simulink model "W06_7_front"  (R2024b)
settings: Solver=ode4  StartTime=0  StopTime=150  FixedStep=h  RelTol=1e-3
InitFcn:
  | addpath(fullfile(fileparts(fileparts(fileparts(get_param(bdroot, 'FileName')))), '_tools'), fileparts(get_param(bdroot, 'FileName'))); run_alone('W06', bdroot);
StopFcn:
  | W06_plot;
values from neighbouring files (symbols this model uses):
  animate = 1    [W06_0_setup.m]    (also in W06_1_point_run.m = 0; W06_2_sway_run.m = 0; W06_3_thrust_run.m = 0; W06_4_stop_run.m = 0)
  berth_E = 1.2    [W06_0_setup.m]
  berth_N = 40    [W06_0_setup.m]
  beta_c = pi/2    (= 1.57079632679)    [W06_0_setup.m]    (also in W06_4_stop_run.m = V.beta_c)
  Binv = inv(B)    [W06_0_setup.m]
  bow = [l_f, k_bow, n_bow_max]    [W06_0_setup.m]
  h = 0.02    [W06_0_setup.m]
  k_bow = cfg.k_bow    [W06_0_setup.m]
  k_neg = cfg.k_neg    [W06_0_setup.m]
  k_pos = cfg.k_pos    [W06_0_setup.m]
  Kb = 1    [W06_0_setup.m]
  Kd = 100    [W06_0_setup.m]
  Ki_u = 200    [W06_0_setup.m]
  Ki_v = 120    [W06_0_setup.m]
  Kp = 300    [W06_0_setup.m]
  Kp_pos = 0.30    (= 0.3)    [W06_0_setup.m]    (also in W06_4_stop_run.m = V.Kp_pos)
  Kp_u = 200    [W06_0_setup.m]
  Kp_v = 150    [W06_0_setup.m]
  mp = 25    [W06_0_setup.m]
  n_bow_max = cfg.n_bow_max    [W06_0_setup.m]    (also in W06_1_point_run.m = V.n_bow_max)
  n_max = cfg.n_max    [W06_0_setup.m]
  N_max = 2*y_pont*min(T_max, -T_min)    [W06_0_setup.m]
  n_min = cfg.n_min    [W06_0_setup.m]
  psi_tol = deg2rad(5)    [W06_0_setup.m]
  R_app = 1.5    [W06_0_setup.m]
  R_berth = 0.40    (= 0.4)    [W06_0_setup.m]
  r_tol = deg2rad(1.0)    [W06_0_setup.m]
  rp = [0.05 0 -0.35]'    [W06_0_setup.m]
  stand_off = 7    [W06_0_setup.m]
  u_lim = 0.80    (= 0.8)    [W06_0_setup.m]
  V_c = 0    [W06_0_setup.m]    (also in W06_4_stop_run.m = V.V_c)
  v_lim = 0.35    [W06_0_setup.m]
  v_tol = 0.05    [W06_0_setup.m]
  x0 = zeros(12,1)    [W06_0_setup.m]
  X_max = 120    [W06_0_setup.m]    (also in W06_plot.m = base_var('X_max', 120))
  Y_max = min(abs(T_min)/(l_f/(2*y_pont)), F_B_max)    [W06_0_setup.m]    (also in W06_plot.m = base_var('Y_max', 35.13))
settings Model: Creator=admin  LastModifiedBy=admin
settings DataIOCC: ReturnWorkspaceOutputs=off

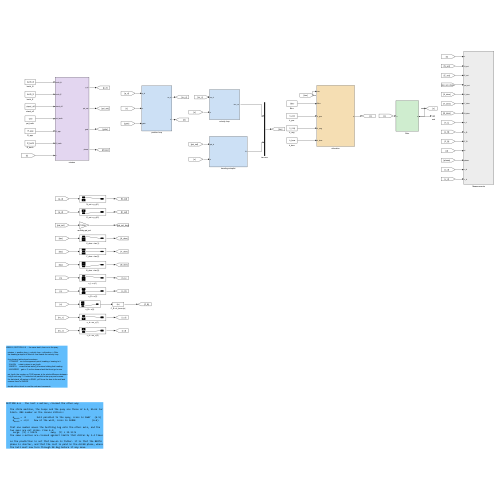
[thumbnail: Simulink's stored preview of the top-level diagram]
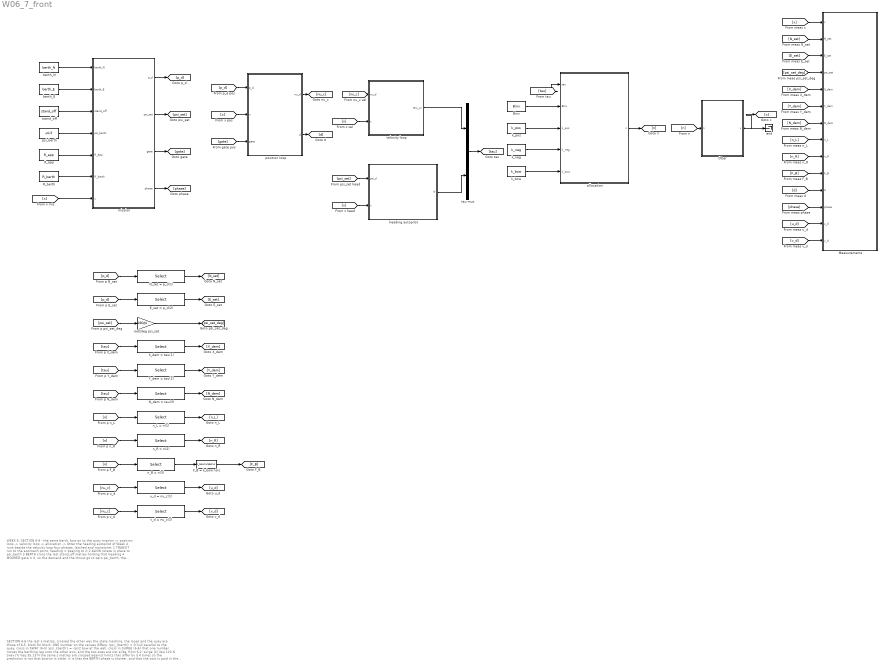
== system W06_7_front ==
  note: WEEK 6, SECTION 6-6  -  the same berth, bow on to the quay
      |
      |    mission -> position loop -> velocity loop -> allocation -> Otter
      |    the heading autopilot of Week 4 runs beside the velocity loop
      |
      |    four phases, latched and monotone:
      |      1 TRANSIT   run to the approach point, heading = bearing to it
      |      2 ALIGN     rotate in place to psi_berth
      |      3 BERTH     cross the last stand_off metres holding that heading
      |      4 MOORED    gate = 0, so the demand and the thrust go to zero
      |
      |    psi_berth, the number on THIS canvas, is the whole difference between
      |    rung 5 and rung 7: 0 holds the hull parallel to the quay and crosses
      |    the last stand_off metres in SWAY, -pi/2 turns the bow to the wall and
      |    crosses them in SURGE
      |
      |    double-click a block to read its code and comments
  note: SECTION 6-6   the last s metres, crossed the other way
      |
      |    the state machine, the loops and the quay are those of 6-5, block for
      |    block. ONE number on the canvas differs:
      |
      |      \psi_{berth} =  0        hull parallel to the quay, cross in SWAY   (6-5)
      |      \psi_{berth} = -\pi/2    bow at the wall, cross in SURGE            (6-6)
      |
      |    that one number moves the berthing leg onto the other axis, and the
      |    two axes are not alike. from 6-2:
      |      surge  |X| \leq 120 N          sway  |Y| \leq 35.13 N
      |    the same s metres are crossed against limits that differ by 3.4 times
      |
      |    so the prediction is not that bow-on is tidier. it is that the BERTH
      |    phase is shorter, and that the cost is paid in the ALIGN phase, where
      |    the hull must now turn through 90 deg before it may move
  Binv : Constant  Value=Binv
  E_set = p_d(2) : Selector  InputPortWidth=2  IndexOptions=Index vector (dialog)  Indices=2  OutputSizes=1
  F_B = k_bow n|n| : Fcn  Expr=k_bow*u*abs(u)
  Measurements : Subsystem
  N_dem = tau(3) : Selector  InputPortWidth=3  IndexOptions=Index vector (dialog)  Indices=3  OutputSizes=1
  N_set = p_d(1) : Selector  InputPortWidth=2  IndexOptions=Index vector (dialog)  Indices=1  OutputSizes=1
  Otter : Subsystem
  R_app : Constant  Value=R_app
  R_berth : Constant  Value=R_berth
  X_dem = tau(1) : Selector  InputPortWidth=3  IndexOptions=Index vector (dialog)  Indices=1  OutputSizes=1
  Y_dem = tau(2) : Selector  InputPortWidth=3  IndexOptions=Index vector (dialog)  Indices=2  OutputSizes=1
  allocation : Subsystem
  berth_E : Constant  Value=berth_E
  berth_N : Constant  Value=berth_N
  end : Terminator
  heading autopilot : Subsystem
  k_bow : Constant  Value=k_bow
  k_neg : Constant  Value=k_neg
  k_pos : Constant  Value=k_pos
  mission : Subsystem
  n_B = n(3) : Selector  InputPortWidth=3  IndexOptions=Index vector (dialog)  Indices=3  OutputSizes=1
  n_L = n(1) : Selector  InputPortWidth=3  IndexOptions=Index vector (dialog)  Indices=1  OutputSizes=1
  n_R = n(2) : Selector  InputPortWidth=3  IndexOptions=Index vector (dialog)  Indices=2  OutputSizes=1
  position loop : Subsystem
  psi_berth : Constant  Value=-pi/2
  rad2deg psi_set : Gain  Gain=180/pi
  stand_off : Constant  Value=stand_off
  tau mux : Mux  Inputs=2
  u_d = nu_c(1) : Selector  InputPortWidth=2  IndexOptions=Index vector (dialog)  Indices=1  OutputSizes=1
  v_d = nu_c(2) : Selector  InputPortWidth=2  IndexOptions=Index vector (dialog)  Indices=2  OutputSizes=1
  velocity loop : Subsystem
  wires:
  berth_N/1 -> mission/1(berth_N)
  berth_E/1 -> mission/2(berth_E)
  stand_off/1 -> mission/3(stand_off)
  psi_berth/1 -> mission/4(psi_berth)
  R_app/1 -> mission/5(R_app)
  R_berth/1 -> mission/6(R_berth)
  [x] -> mission/7(x)
  mission/1(p_d) -> [p_d]
  mission/2(psi_set) -> [psi_set]
  mission/3(gate) -> [gate]
  mission/4(phase) -> [phase]
  [p_d] -> position loop/1(p_d)
  [x] -> position loop/2(x)
  [gate] -> position loop/3(gate)
  position loop/2(d) -> [d]
  position loop/1(nu_d) -> [nu_c]
  [nu_c] -> velocity loop/1(nu_d)
  [x] -> velocity loop/2(x)
  [psi_set] -> heading autopilot/1(psi_d)
  [x] -> heading autopilot/2(x)
  velocity loop/1(tau_uv) -> tau mux/1
  heading autopilot/1(N) -> tau mux/2
  tau mux/1 -> [tau]
  [tau] -> allocation/1(tau)
  Binv/1 -> allocation/2(Binv)
  k_pos/1 -> allocation/3(k_pos)
  k_neg/1 -> allocation/4(k_neg)
  k_bow/1 -> allocation/5(k_bow)
  allocation/1(n) -> [n]
  [n] -> Otter/1(n)
  Otter/1(x) -> [x], end/1
  [x] -> Measurements/1(x)
  [N_set] -> Measurements/2(N_set)
  [E_set] -> Measurements/3(E_set)
  [psi_set_deg] -> Measurements/4(psi_set)
  [X_dem] -> Measurements/5(X_dem)
  [Y_dem] -> Measurements/6(Y_dem)
  [N_dem] -> Measurements/7(N_dem)
  [n_L] -> Measurements/8(n_L)
  [n_R] -> Measurements/9(n_R)
  [F_B] -> Measurements/10(F_B)
  [d] -> Measurements/11(d)
  [phase] -> Measurements/12(phase)
  [u_d] -> Measurements/13(u_d)
  [v_d] -> Measurements/14(v_d)
  [p_d] -> N_set = p_d(1)/1
  N_set = p_d(1)/1 -> [N_set]
  [p_d] -> E_set = p_d(2)/1
  E_set = p_d(2)/1 -> [E_set]
  [psi_set] -> rad2deg psi_set/1
  rad2deg psi_set/1 -> [psi_set_deg]
  [tau] -> X_dem = tau(1)/1
  X_dem = tau(1)/1 -> [X_dem]
  [tau] -> Y_dem = tau(2)/1
  Y_dem = tau(2)/1 -> [Y_dem]
  [tau] -> N_dem = tau(3)/1
  N_dem = tau(3)/1 -> [N_dem]
  [n] -> n_L = n(1)/1
  n_L = n(1)/1 -> [n_L]
  [n] -> n_R = n(2)/1
  n_R = n(2)/1 -> [n_R]
  [n] -> n_B = n(3)/1
  n_B = n(3)/1 -> F_B = k_bow n|n|/1
  F_B = k_bow n|n|/1 -> [F_B]
  [nu_c] -> u_d = nu_c(1)/1
  u_d = nu_c(1)/1 -> [u_d]
  [nu_c] -> v_d = nu_c(2)/1
  v_d = nu_c(2)/1 -> [v_d]

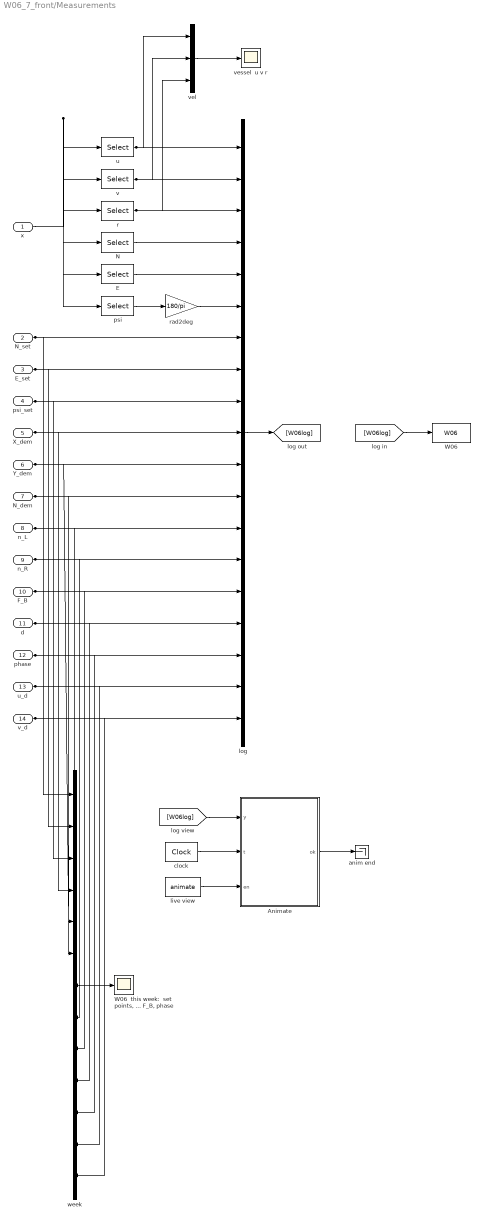
== system W06_7_front/Measurements ==
  x : Inport
  N_set : Inport  Port=2
  E_set : Inport  Port=3
  psi_set : Inport  Port=4
  X_dem : Inport  Port=5
  Y_dem : Inport  Port=6
  N_dem : Inport  Port=7
  n_L : Inport  Port=8
  n_R : Inport  Port=9
  F_B : Inport  Port=10
  d : Inport  Port=11
  phase : Inport  Port=12
  u_d : Inport  Port=13
  v_d : Inport  Port=14
  Animate : MATLAB Function  TreatAsAtomicUnit=on
  E : Selector  InputPortWidth=12  IndexOptions=Index vector (dialog)  Indices=8  OutputSizes=1
  N : Selector  InputPortWidth=12  IndexOptions=Index vector (dialog)  Indices=7  OutputSizes=1
  W06 : ToWorkspace  VariableName=W06  SaveFormat=Structure With Time  SampleTime=-1
  "W06  this week:  set points, demands, n_L n_R, F_B, phase" : Scope
  anim end : Terminator
  clock : DigitalClock  SampleTime=h
  live view : Constant  Value=animate
  log : Mux  Inputs=19
  psi : Selector  InputPortWidth=12  IndexOptions=Index vector (dialog)  Indices=12  OutputSizes=1
  r : Selector  InputPortWidth=12  IndexOptions=Index vector (dialog)  Indices=6  OutputSizes=1
  rad2deg : Gain  Gain=180/pi
  u : Selector  InputPortWidth=12  IndexOptions=Index vector (dialog)  Indices=1  OutputSizes=1
  v : Selector  InputPortWidth=12  IndexOptions=Index vector (dialog)  Indices=2  OutputSizes=1
  vel : Mux  Inputs=3
  vessel  u v r : Scope
  week : Mux  Inputs=13
  wires:
  x/1 -> u/1, v/1, r/1, N/1, E/1, psi/1
  log/1 -> [W06log]
  [W06log] -> W06/1
  psi/1 -> rad2deg/1
  u/1 -> log/1, vel/1
  v/1 -> log/2, vel/2
  r/1 -> log/3, vel/3
  N/1 -> log/4
  E/1 -> log/5
  rad2deg/1 -> log/6
  N_set/1 -> log/7, week/1
  E_set/1 -> log/8, week/2
  psi_set/1 -> log/9, week/3
  X_dem/1 -> log/10, week/4
  Y_dem/1 -> log/11, week/5
  N_dem/1 -> log/12, week/6
  n_L/1 -> log/13, week/7
  n_R/1 -> log/14, week/8
  F_B/1 -> log/15, week/9
  d/1 -> log/16, week/10
  phase/1 -> log/17, week/11
  u_d/1 -> log/18, week/12
  v_d/1 -> log/19, week/13
  vel/1 -> vessel  u v r/1
  week/1 -> "W06  this week:  set points, demands, n_L n_R, F_B, phase"/1
  [W06log] -> Animate/1(y)
  clock/1 -> Animate/2(t)
  live view/1 -> Animate/3(en)
  Animate/1(ok) -> anim end/1

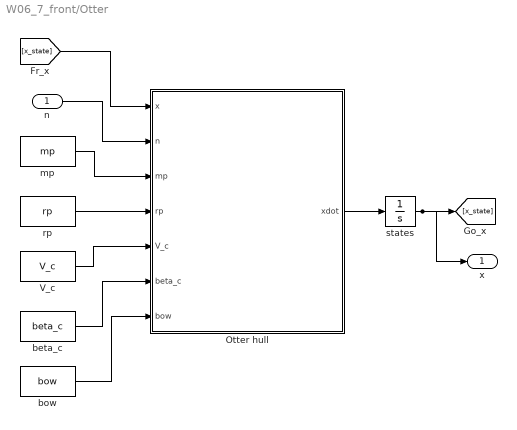
== system W06_7_front/Otter ==
  n : Inport
  Otter hull : MATLAB Function  TreatAsAtomicUnit=on
  V_c : Constant  Value=V_c
  beta_c : Constant  Value=beta_c
  bow : Constant  Value=bow
  mp : Constant  Value=mp
  rp : Constant  Value=rp
  states : Integrator  InitialCondition=x0
  x : Outport
  wires:
  [x_state] -> Otter hull/1(x)
  rp/1 -> Otter hull/4(rp)
  bow/1 -> Otter hull/7(bow)
  n/1 -> Otter hull/2(n)
  mp/1 -> Otter hull/3(mp)
  V_c/1 -> Otter hull/5(V_c)
  beta_c/1 -> Otter hull/6(beta_c)
  Otter hull/1(xdot) -> states/1
  states/1 -> [x_state], x/1

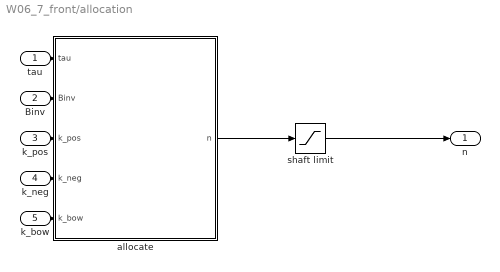
== system W06_7_front/allocation ==
  tau : Inport
  Binv : Inport  Port=2
  k_pos : Inport  Port=3
  k_neg : Inport  Port=4
  k_bow : Inport  Port=5
  allocate : MATLAB Function  TreatAsAtomicUnit=on
  shaft limit : Saturate  UpperLimit="[ n_max;  n_max;  n_bow_max]"  LowerLimit="[ n_min;  n_min; -n_bow_max]"
  n : Outport
  wires:
  tau/1 -> allocate/1(tau)
  Binv/1 -> allocate/2(Binv)
  k_pos/1 -> allocate/3(k_pos)
  k_neg/1 -> allocate/4(k_neg)
  k_bow/1 -> allocate/5(k_bow)
  allocate/1(n) -> shaft limit/1
  shaft limit/1 -> n/1

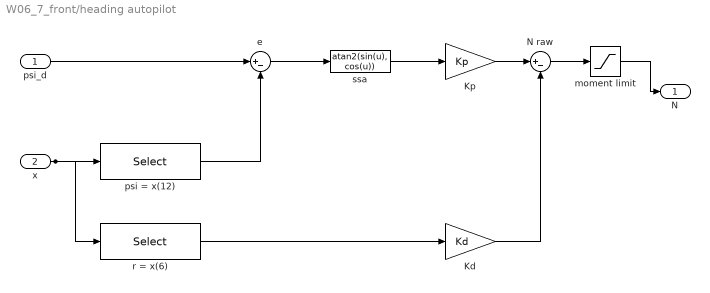
== system W06_7_front/heading autopilot ==
  psi_d : Inport
  x : Inport  Port=2
  Kd : Gain  Gain=Kd
  Kp : Gain  Gain=Kp
  N raw : Sum  Inputs=|+-
  e : Sum  Inputs=|+-
  moment limit : Saturate  UpperLimit=N_max  LowerLimit=-N_max
  psi = x(12) : Selector  InputPortWidth=12  IndexOptions=Index vector (dialog)  Indices=12  OutputSizes=1
  r = x(6) : Selector  InputPortWidth=12  IndexOptions=Index vector (dialog)  Indices=6  OutputSizes=1
  ssa : Fcn  Expr=atan2(sin(u), cos(u))
  N : Outport
  wires:
  x/1 -> psi = x(12)/1, r = x(6)/1
  psi_d/1 -> e/1
  psi = x(12)/1 -> e/2
  e/1 -> ssa/1
  ssa/1 -> Kp/1
  r = x(6)/1 -> Kd/1
  Kp/1 -> N raw/1
  Kd/1 -> N raw/2
  N raw/1 -> moment limit/1
  moment limit/1 -> N/1

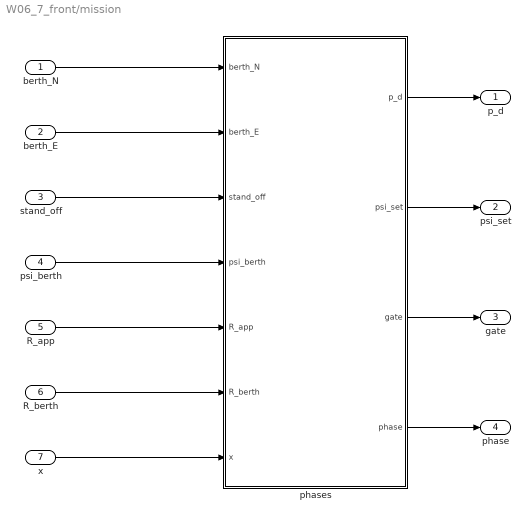
== system W06_7_front/mission ==
  berth_N : Inport
  berth_E : Inport  Port=2
  stand_off : Inport  Port=3
  psi_berth : Inport  Port=4
  R_app : Inport  Port=5
  R_berth : Inport  Port=6
  x : Inport  Port=7
  phases : MATLAB Function  TreatAsAtomicUnit=on
  p_d : Outport
  psi_set : Outport  Port=2
  gate : Outport  Port=3
  phase : Outport  Port=4
  wires:
  berth_N/1 -> phases/1(berth_N)
  berth_E/1 -> phases/2(berth_E)
  stand_off/1 -> phases/3(stand_off)
  psi_berth/1 -> phases/4(psi_berth)
  R_app/1 -> phases/5(R_app)
  R_berth/1 -> phases/6(R_berth)
  x/1 -> phases/7(x)
  phases/1(p_d) -> p_d/1
  phases/2(psi_set) -> psi_set/1
  phases/3(gate) -> gate/1
  phases/4(phase) -> phase/1

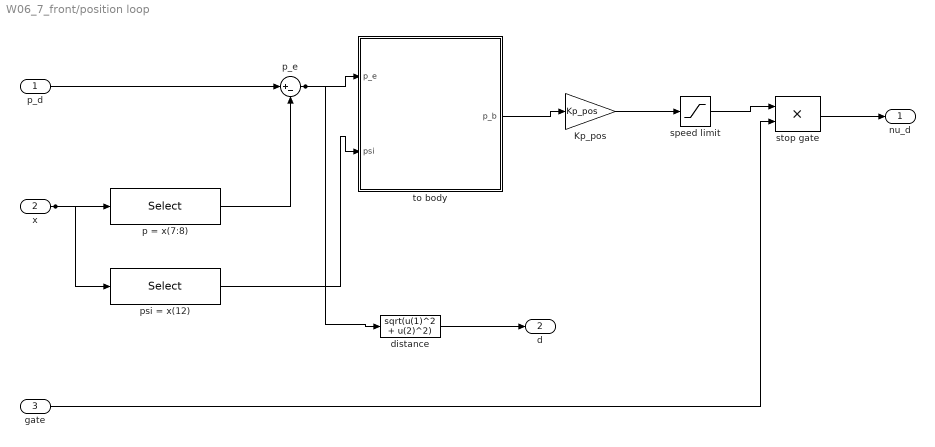
== system W06_7_front/position loop ==
  p_d : Inport
  x : Inport  Port=2
  gate : Inport  Port=3
  Kp_pos : Gain  Gain=Kp_pos
  distance : Fcn  Expr=sqrt(u(1)^2 + u(2)^2)
  p = x(7:8) : Selector  InputPortWidth=12  IndexOptions=Index vector (dialog)  Indices=[7 8]  OutputSizes=1
  p_e : Sum  Inputs=|+-
  psi = x(12) : Selector  InputPortWidth=12  IndexOptions=Index vector (dialog)  Indices=12  OutputSizes=1
  speed limit : Saturate  UpperLimit="[ u_lim;  v_lim]"  LowerLimit=[-u_lim; -v_lim]
  stop gate : Product
  to body : MATLAB Function  TreatAsAtomicUnit=on
  nu_d : Outport
  d : Outport  Port=2
  wires:
  x/1 -> p = x(7:8)/1, psi = x(12)/1
  p_d/1 -> p_e/1
  p = x(7:8)/1 -> p_e/2
  p_e/1 -> to body/1(p_e), distance/1
  psi = x(12)/1 -> to body/2(psi)
  to body/1(p_b) -> Kp_pos/1
  Kp_pos/1 -> speed limit/1
  speed limit/1 -> stop gate/1
  gate/1 -> stop gate/2
  stop gate/1 -> nu_d/1
  distance/1 -> d/1

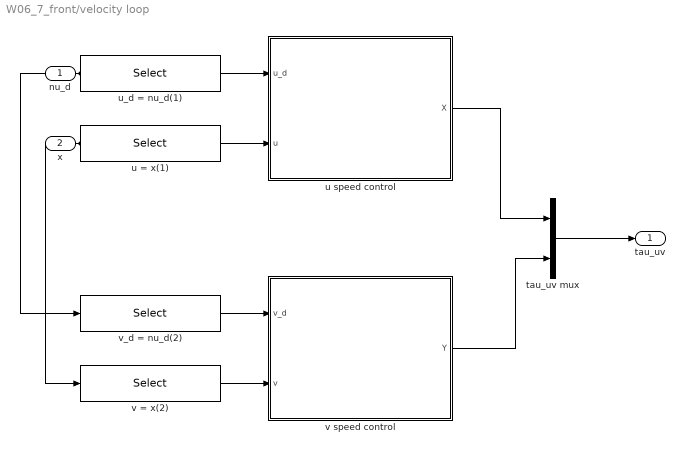
== system W06_7_front/velocity loop ==
  nu_d : Inport
  x : Inport  Port=2
  tau_uv mux : Mux  Inputs=2
  u = x(1) : Selector  InputPortWidth=12  IndexOptions=Index vector (dialog)  Indices=1  OutputSizes=1
  u speed control : Subsystem
  u_d = nu_d(1) : Selector  InputPortWidth=2  IndexOptions=Index vector (dialog)  Indices=1  OutputSizes=1
  v = x(2) : Selector  InputPortWidth=12  IndexOptions=Index vector (dialog)  Indices=2  OutputSizes=1
  v speed control : Subsystem
  v_d = nu_d(2) : Selector  InputPortWidth=2  IndexOptions=Index vector (dialog)  Indices=2  OutputSizes=1
  tau_uv : Outport
  wires:
  u_d = nu_d(1)/1 -> u speed control/1(u_d)
  u = x(1)/1 -> u speed control/2(u)
  v_d = nu_d(2)/1 -> v speed control/1(v_d)
  v = x(2)/1 -> v speed control/2(v)
  nu_d/1 -> u_d = nu_d(1)/1, v_d = nu_d(2)/1
  x/1 -> u = x(1)/1, v = x(2)/1
  u speed control/1(X) -> tau_uv mux/1
  v speed control/1(Y) -> tau_uv mux/2
  tau_uv mux/1 -> tau_uv/1

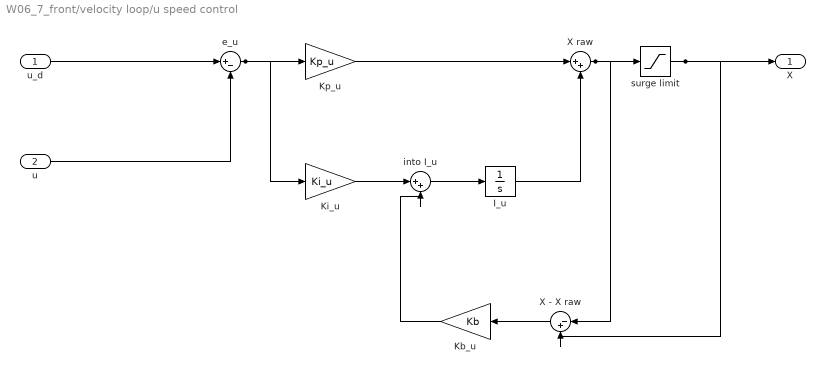
== system W06_7_front/velocity loop/u speed control ==
  u_d : Inport
  u : Inport  Port=2
  I_u : Integrator
  Kb_u : Gain  Gain=Kb
  Ki_u : Gain  Gain=Ki_u
  Kp_u : Gain  Gain=Kp_u
  X - X raw : Sum  Inputs=|-+
  X raw : Sum  Inputs=|++
  e_u : Sum  Inputs=|+-
  into I_u : Sum  Inputs=|++
  surge limit : Saturate  UpperLimit=X_max  LowerLimit=-X_max
  X : Outport
  wires:
  u_d/1 -> e_u/1
  u/1 -> e_u/2
  e_u/1 -> Kp_u/1, Ki_u/1
  Ki_u/1 -> into I_u/1
  into I_u/1 -> I_u/1
  Kp_u/1 -> X raw/1
  I_u/1 -> X raw/2
  X raw/1 -> surge limit/1, X - X raw/1
  surge limit/1 -> X - X raw/2, X/1
  X - X raw/1 -> Kb_u/1
  Kb_u/1 -> into I_u/2

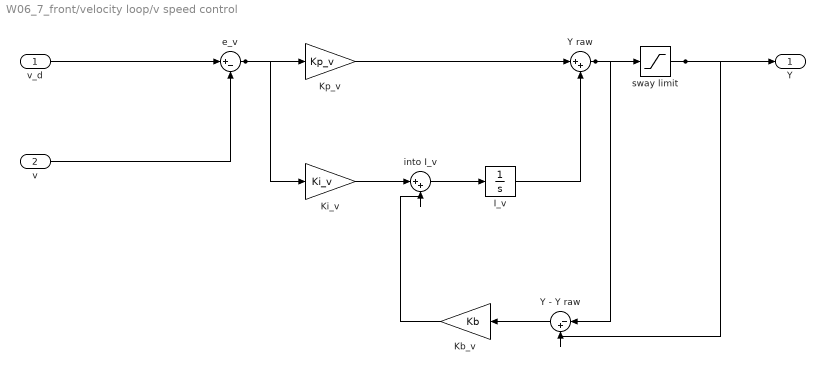
== system W06_7_front/velocity loop/v speed control ==
  v_d : Inport
  v : Inport  Port=2
  I_v : Integrator
  Kb_v : Gain  Gain=Kb
  Ki_v : Gain  Gain=Ki_v
  Kp_v : Gain  Gain=Kp_v
  Y - Y raw : Sum  Inputs=|-+
  Y raw : Sum  Inputs=|++
  e_v : Sum  Inputs=|+-
  into I_v : Sum  Inputs=|++
  sway limit : Saturate  UpperLimit=Y_max  LowerLimit=-Y_max
  Y : Outport
  wires:
  v_d/1 -> e_v/1
  v/1 -> e_v/2
  e_v/1 -> Kp_v/1, Ki_v/1
  Ki_v/1 -> into I_v/1
  into I_v/1 -> I_v/1
  Kp_v/1 -> Y raw/1
  I_v/1 -> Y raw/2
  Y raw/1 -> sway limit/1, Y - Y raw/1
  sway limit/1 -> Y - Y raw/2, Y/1
  Y - Y raw/1 -> Kb_v/1
  Kb_v/1 -> into I_v/2

== matlab function W06_7_front/position loop/to body ==
  data: p_e input; p_b output double size=[2 1]; psi input
function p_b = to_body(p_e, psi)
% Rotate the position error from NED into the body frame.
%
%            [ cos(psi)  -sin(psi) ]
%   R(psi) = [ sin(psi)   cos(psi) ]     maps the BODY frame to NED,
%
% so the transpose maps NED to the body frame. R is orthogonal, so the
% transpose is the inverse and nothing is lost in the change of frame: the
% distance to the target is the same number in either one.
c = cos(psi);
s = sin(psi);
p_b = [  c*p_e(1) + s*p_e(2) ;      % 전진 방향의 오차 / along the bow
        -s*p_e(1) + c*p_e(2) ];     % 우현 방향의 오차 / to starboard
end

== matlab function W06_7_front/mission/phases ==
  settings: updateMethod=DISCRETE  sampleTime=h
  data: berth_N input; p_d output double size=[2 1]; berth_E input; stand_off input; psi_berth input; R_app input; R_berth input; x input; psi_set output; gate output; phase output; psi_tol parameter; v_tol parameter; r_tol parameter
function [p_d, psi_set, gate, phase] = phases(berth_N, berth_E, stand_off, ...
                                                psi_berth, R_app, R_berth, x, ...
                                                psi_tol, v_tol, r_tol)
%#codegen
%  네 단계. 한 번 넘어가면 돌아오지 않는다 — 빗장이 걸려 있다.
%  Four phases. Once a transition is taken it is never taken back: it latches.
%
%    1 TRANSIT  접근점으로 간다. 선수각은 그쪽 방위 (5주차의 atan2 법칙)
%    2 ALIGN    제자리에서 psi_berth 로 돌린다
%    3 BERTH    그 선수각을 지킨 채 남은 stand_off 미터를 간다
%    4 MOORED   gate = 0 — 계류줄이 걸렸고 추진기는 0 으로 간다
%
%  왜 빗장을 거는가 / why it latches
%      단계마다 조건이 **경계에서** 참과 거짓을 왕복한다. 빗장이 없으면 배가
%      반경 R_app 안팎을 드나들 때 목표점이 접근점과 접안점 사이를 떨고,
%      안쪽 루프는 그 떨림을 추력으로 바꾼다.
%      Each condition flickers at its own boundary. Without the latch the
%      target would jitter between the two points and the inner loops would
%      turn that jitter into thrust.
%
%  왜 선수각을 **들고 있는가** / why the heading is HELD
%      1 단계의 선수각은 접근점 방위다. 접근점에 가까워지면 그 방위의 분모가
%      0 으로 가므로 2 m 안에서는 **마지막 값을 들고 있는다**. 이것이 이 절이
%      재는 예측 하나를 만든다 — 명령 선수각이 그 시각부터 평평해진다.
%      The bearing is ill-conditioned near the point, so inside 2 m the last
%      value is held. This section measures the prediction that makes: the
%      commanded heading goes flat from that instant.

persistent ph psi_hold
if isempty(ph), ph = 1; psi_hold = x(12); end

p   = [x(7); x(8)];     %  NED 위치 / position in NED
psi = x(12);
r   = x(6);
v   = x(2);

app = [berth_N; berth_E + stand_off];   %  접근점 / the approach point
brt = [berth_N; berth_E];               %  접안점 / the berth

switch ph
    case 1      %  TRANSIT
        e = app - p;
        if norm(e) > 2
            psi_hold = atan2(e(2), e(1));
        end
        if norm(e) <= R_app, ph = 2; end

    case 2      %  ALIGN
        psi_hold = psi_berth;
        de = atan2(sin(psi - psi_berth), cos(psi - psi_berth));
        if abs(de) <= psi_tol && abs(r) <= r_tol, ph = 3; end

    case 3      %  BERTH
        psi_hold = psi_berth;
        if norm(brt - p) <= R_berth && abs(v) <= v_tol, ph = 4; end

    otherwise   %  MOORED
        psi_hold = psi_berth;
end

if ph >= 3
    p_d = brt;
else
    p_d = app;
end
psi_set = psi_hold;
gate    = double(ph <= 3);   %  4 단계에서 0 — 추력을 끊는다 / thrust off
phase   = ph;
end

== matlab function W06_7_front/allocation/allocate ==
  data: tau input; n output double size=[3 1]; Binv input; k_pos input; k_neg input; k_bow input
function n = allocate(tau, Binv, k_pos, k_neg, k_bow)
% Run the actuator model backwards: tau -> f -> u -> n.
%
%   forward    u_i = n_i|n_i|      f = K u        tau = B f
%   inverse    f = B^-1 tau        u = K^-1 f     n_i = sign(u_i) sqrt(|u_i|)
%
%   B    = [    1         1       0  ]    f   = [T_L; T_R; F_B]  [N]
%          [    0         0       1  ]    tau = [X; Y; N]        [N, N, N m]
%          [ y_pont   -y_pont   l_f ]
%
% B is square and non-singular (det B = 0.79), so the solution is unique and
% there is no null space to choose within. Binv comes from the setup script,
% which inverts the B that otter_B() derives from the column rule.
f = Binv * tau;

% K is diagonal, so K^-1 is three divisions. Which coefficient applies depends
% on the sign for a stern propeller, because a propeller pushing astern is
% less efficient than the same propeller pushing ahead. It does not depend on
% the sign for the bow unit: a tunnel thruster is symmetric.
k = [k_pos; k_pos; k_bow];
if f(1) < 0, k(1) = k_neg; end
if f(2) < 0, k(2) = k_neg; end

u = f ./ k;

% n_i = sign(u_i) sqrt(|u_i|). The absolute value is not decoration: slide 133
% writes sqrt(u_i), and without the |.| every astern command returns a complex
% shaft speed.
n = sign(u) .* sqrt(abs(u));
end

== matlab function W06_7_front/Otter/Otter hull ==
  data: x input; xdot output double size=[12 1]; n input; mp input; rp input; V_c input; beta_c input; bow input
function xdot = otter_hull(x, n, mp, rp, V_c, beta_c, bow)
% otter_bow.m: Fossen's otter.m with a bow tunnel thruster added, called
% unchanged from _tools. Three shaft speeds in, tau built inside.
%
%   x     12 states, fed back from the integrator
%   n     shaft speeds [rad/s]: port stern, starboard stern, bow
%   bow   [l3 k3 n3_max], the bow unit's arm, coefficient and speed limit
%
% The sway force and its moment are now rows 2 and 6 of the tau that the
% motion model builds for itself. Nothing is added after the call.
%
% otter_bow.m is not written for code generation, so the call is extrinsic
% and xdot has to be pre-sized for Simulink to know the output width.
coder.extrinsic('otter_bow');

xdot = zeros(12,1);
xdot = otter_bow(x, n, mp, rp, V_c, beta_c, bow);
end

== matlab function W06_7_front/Measurements/Animate ==
  data: y input; ok output; t input; en input
function ok = Animate(y, t, en)
%#codegen
% Live view of the vessel while the model runs.
%
% A MATLAB Function block cannot plot, so the drawing function is declared
% extrinsic: Simulink calls plain MATLAB rather than generating code for it.
% Set animate = 0 in the setup script to switch the live view off.
%
% y is the whole log vector, in the column order this subsystem builds:
% [u v r N E psi] first, psi in DEGREES, then the week's own signals.
% The wrapper names the columns; nothing else counts them.
coder.extrinsic('W06_animate');
ok = 1;
if en > 0.5
    W06_animate(y, t);
end
end
